simulink model "diagram"  (R2025a)
settings: Solver=VariableStepAuto  StartTime=0.0  StopTime=10.0  RelTol=1e-3
values from neighbouring files (symbols this model uses):
  J = 0.05    [init_pmsm_params.m]    (also in matlab.mat = 0.02)
  Kd_i = 0.01    [matlab.mat]
  Kd_omega = 1    [matlab.mat]
  Kd_theta = 1    [matlab.mat]
  Ke = 0.023    [matlab.mat]
  Kp_i = 2    [matlab.mat]
  Kp_omega = 10    [matlab.mat]
  Kp_theta = 15    [matlab.mat]
  Kt = 0.023    [matlab.mat]
  L = 0.0023    [matlab.mat]
  R = 2    [matlab.mat]
settings Model: Creator=frf  LastModifiedBy=frf

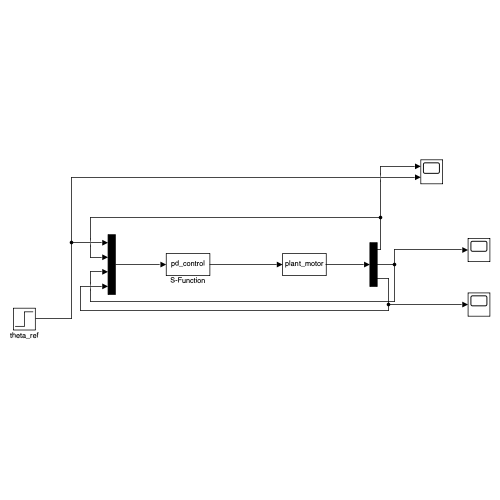
[thumbnail: Simulink's stored preview of the top-level diagram]
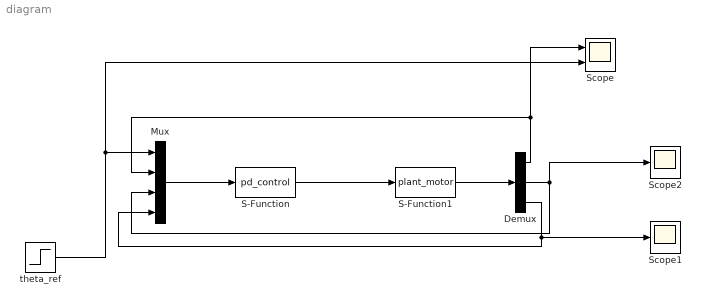
== system diagram ==
  Demux : Demux  Outputs=3
  Mux : Mux
  S-Function : S-Function  FunctionName=pd_control  Parameters=[Kp_theta], [Kd_theta], [Kp_omega], [Kd_omega], [Kp_i], [Kd_i]  SFunctionDeploymentMode=off  EnableBusSupport=off
  S-Function1 : S-Function  FunctionName=plant_motor  Parameters=[J], [Kt], [Ke], [R], [L]  SFunctionDeploymentMode=off  EnableBusSupport=off
  Scope : Scope  NumInputPorts=2
      settings: ActiveDisplayYMinimum=-0.69353398416148182  ActiveDisplayYMaximum=1.5585527805092572
  Scope1 : Scope
  Scope2 : Scope
      settings: DataLoggingVariableName=ScopeData2
  theta_ref : Step  SampleTime=0
  wires:
  S-Function/1 -> S-Function1/1
  S-Function1/1 -> Demux/1
  theta_ref/1 -> Scope/2, Mux/1
  Mux/1 -> S-Function/1
  Demux/1 -> Mux/2, Scope/1
  Demux/2 -> Scope2/1, Mux/3
  Demux/3 -> Mux/4, Scope1/1
